simulink model "sistema"  (R2026a)
settings: Solver=ode15s  MaxStep=1E-3
libraries: fl_lib x14, nesl_utility x6, slpidlib x1
settings Model: LastModifiedBy=Mariant Javtech
settings DataIOCC: TimeSaveName=t
settings DebuggingCC: ArtificialAlgebraicLoopMsg=none  MaxConsecutiveZCsMsg=none  OperatingPointInterfaceChecksumMismatchMsg=none
settings SimscapeCC: SimscapeNominalValues="[{\"value\":\"1\",\"unit\":\"A\"},{\"value\":\"1\",\"unit\":\"bar\"},{\"value\":\"1\",\"unit\":\"cm^2\"},{\"value\":\"1\",\"unit\":\"cm^3/s\"},{\"value\":\"1\",\"unit\":\"kJ/kg\"},{\"value\":\"1\",\"unit\":\"kW\"},{\"value\":\"1\",\"unit\":\"l\"},{\"value\":\"1\",\"unit\":\"N\"},{\"value\":\"1\",\"unit\":\"N*m\"},{\"value\":\"1\",\"unit\":\"V\"}]"  SimscapeLogType=none  SimscapeLogDataHistory=5000.0

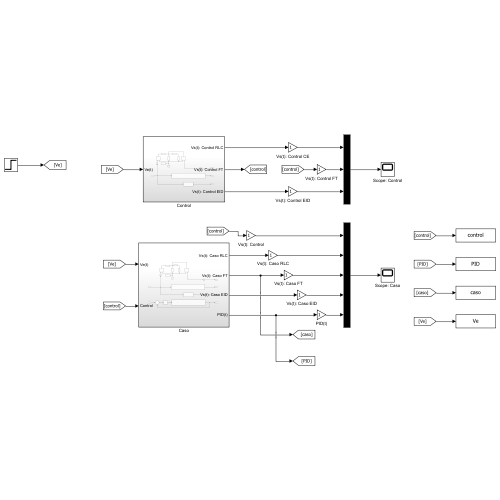
[thumbnail: Simulink's stored preview of the top-level diagram]
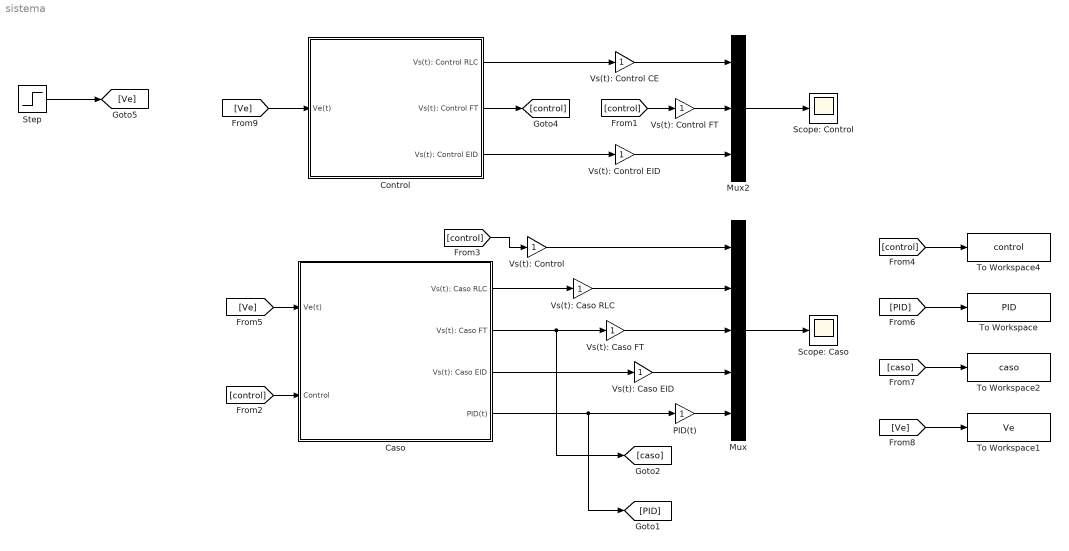
== system sistema ==
  Caso : Subsystem
  Control : Subsystem
  Mux : Mux  Inputs=5
  Mux2 : Mux  Inputs=3
  PID(t) : Gain
  Scope: Caso : Scope
      settings: ActiveDisplayYMinimum=-0.13044665193336266  ActiveDisplayYMaximum=1.1740198674002642
  Scope: Control : Scope
      settings: ActiveDisplayYMinimum=-0.13608  ActiveDisplayYMaximum=1.22472  DataLoggingVariableName=ScopeData2
  Step : Step  Time=0  SampleTime=0
  To Workspace : ToWorkspace  VariableName=PID  SampleTime=-1
  To Workspace1 : ToWorkspace  VariableName=Ve  SampleTime=-1
  To Workspace2 : ToWorkspace  VariableName=caso  SampleTime=-1
  To Workspace4 : ToWorkspace  VariableName=control  SampleTime=-1
  Vs(t): Caso EID : Gain
  Vs(t): Caso FT : Gain
  Vs(t): Caso RLC : Gain
  Vs(t): Control : Gain
  Vs(t): Control CE : Gain
  Vs(t): Control EID : Gain
  Vs(t): Control FT : Gain
  wires:
  Mux/1 -> Scope: Caso/1
  [control] -> Caso/2(Control)
  [control] -> Vs(t): Control/1
  [Ve] -> Caso/1(Ve(t))
  Control/2(Vs(t): Control FT) -> [control]
  Control/1(Vs(t): Control RLC) -> Vs(t): Control CE/1
  Mux2/1 -> Scope: Control/1
  [Ve] -> Control/1(Ve(t))
  Step/1 -> [Ve]
  Vs(t): Control CE/1 -> Mux2/1
  Vs(t): Caso RLC/1 -> Mux/2
  Vs(t): Caso FT/1 -> Mux/3
  [control] -> Vs(t): Control FT/1
  Vs(t): Control FT/1 -> Mux2/2
  Control/3(Vs(t): Control EID) -> Vs(t): Control EID/1
  Vs(t): Control EID/1 -> Mux2/3
  Caso/4(PID(t)) -> [PID], PID(t)/1
  Caso/1(Vs(t): Caso RLC) -> Vs(t): Caso RLC/1
  Caso/2(Vs(t): Caso FT) -> [caso], Vs(t): Caso FT/1
  PID(t)/1 -> Mux/5
  Caso/3(Vs(t): Caso EID) -> Vs(t): Caso EID/1
  Vs(t): Caso EID/1 -> Mux/4
  Vs(t): Control/1 -> Mux/1
  [control] -> To Workspace4/1
  [PID] -> To Workspace/1
  [caso] -> To Workspace2/1
  [Ve] -> To Workspace1/1

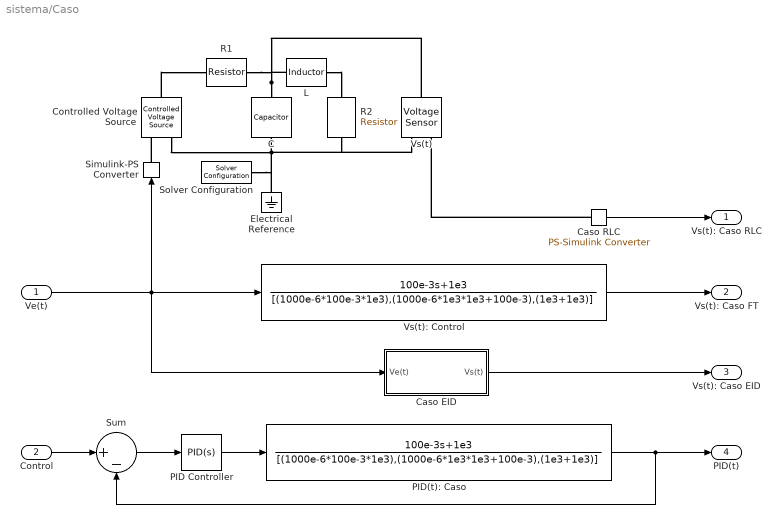
== system sistema/Caso ==
  Ve(t) : Inport
  Control : Inport  Port=2
  C : fl_lib/Electrical/Electrical Elements/Capacitor  c=1000e-6 F  r=1e-6 Ohm  g=0 1/Ohm  i_specify=off  i_priority=None  i=0 A  i_nominal_specify=off  i_nominal_value=1  i_nominal_unit=A  v_specify=off  v_priority=None  v=0 V  v_nominal_specify=off  v_nominal_value=1  v_nominal_unit=V  vc_specify=off  vc_priority=High  vc=0 V  vc_nominal_specify=off  vc_nominal_value=1  vc_nominal_unit=V
  Caso EID : Subsystem
  Caso RLC : nesl_utility/PS-Simulink Converter  PhysicalDomain=network_engine_domain  SubClassName=ps_output  LeftPortType=input  RightPortType=output  PseudoPeriodic=off  Frequencies=[]  VectorFormat=1-D array  Unit=inherit  AffineConversion=off
  Controlled Voltage Source : fl_lib/Electrical/Electrical Sources/Controlled Voltage Source
  Electrical Reference : fl_lib/Electrical/Electrical Elements/Electrical Reference
  L : fl_lib/Electrical/Electrical Elements/Inductor  l=100e-3 H  r=0 Ohm  g=1e-9 1/Ohm  i_specify=off  i_priority=None  i=0 A  i_nominal_specify=off  i_nominal_value=1  i_nominal_unit=A  v_specify=off  v_priority=None  v=0 V  v_nominal_specify=off  v_nominal_value=1  v_nominal_unit=V  i_L_specify=off  i_L_priority=High  i_L=0 A  i_L_nominal_specify=off  i_L_nominal_value=1  i_L_nominal_unit=A
  PID Controller : slpidlib/PID Controller  Controller=PID  Form=Parallel  TimeDomain=Continuous-time  UseExternalTs=off  SampleTime=-1  IntegratorMethod=Forward Euler  FilterMethod=Forward Euler  ControllerParametersSource=internal  P=2048.14768883037  I=776909.685302916  UseKiTs=off  D=0.181141069703887  UseExternalDerivativeSource=off  N=7831.7903058867  UseFilter=on  TunerSelectOption=Transfer Function Based (PID Tuner App)  InitialConditionSource=internal  InitialConditionForIntegrator=0  InitialConditionForFilter=0  DifferentiatorICPrevScaledInput=0  ExternalReset=none  TrackingMode=off  Kt=1  LimitOutput=off  SatLimitsSource=internal  UpperSaturationLimit=inf  LowerSaturationLimit=-inf  LinearizeAsGain=on  AntiWindupMode=none  Kb=1  LimitIntegrator=off  UpperIntegratorSaturationLimit=inf  LowerIntegratorSaturationLimit=-inf  POutMin=[]  POutMax=[]  IOutMin=[]  IOutMax=[]  DOutMin=[]  DOutMax=[]  NOutMin=[]  NOutMax=[]  SumOutMin=[]  SumOutMax=[]  SaturationOutMin=[]  SaturationOutMax=[]  PParamMin=[]  PParamMax=[]  IParamMin=[]  IParamMax=[]  DParamMin=[]  DParamMax=[]  NParamMin=[]  NParamMax=[]  KbParamMin=[]  KbParamMax=[]  KtParamMin=[]  KtParamMax=[]  KbOutMin=[]  KbOutMax=[]  KtOutMin=[]  KtOutMax=[]  IntegratorOutMin=[]  IntegratorOutMax=[]  FilterOutMin=[]  FilterOutMax=[]  SumI1OutMin=[]  SumI1OutMax=[]  SumI2OutMin=[]  SumI2OutMax=[]  SumI3OutMin=[]  SumI3OutMax=[]  SumI4OutMin=[]  SumI4OutMax=[]  SumDOutMin=[]  SumDOutMax=[]  DifferentiatorOutMin=[]  DifferentiatorOutMax=[]  FilterDiffOutCoefMin=[]  FilterDiffOutCoefMax=[]  ReciprocalOutMin=[]  ReciprocalOutMax=[]  SumDenOutMin=[]  SumDenOutMax=[]  SumNumOutMin=[]  SumNumOutMax=[]  DivideOutMin=[]  DivideOutMax=[]  UdiffTsProdOutMin=[]  UdiffTsProdOutMax=[]  NTsProdOutMin=[]  NTsProdOutMax=[]  UintegralTsProdOutMin=[]  UintegralTsProdOutMax=[]  UngainTsProdOutMin=[]  UngainTsProdOutMax=[]  ClampingZeroOutDataTypeStr=Inherit: Inherit via back propagation  ClampingZeroOutMin=[]  ClampingZeroOutMax=[]  FilterDenConstantOutDataTypeStr=Inherit: Inherit via back propagation  FilterDenConstantOutMin=[]  FilterDenConstantOutMax=[]  PCopyOutDataTypeStr=Inherit: Inherit via back propagation  PCopyOutMin=[]  PCopyOutMax=[]  NCopyOutDataTypeStr=Inherit: Inherit via back propagation  NCopyOutMin=[]  NCopyOutMax=[]  IntegratorContinuousStateAttributes=''  IntegratorStateMustResolveToSignalObject=off  IntegratorRTWStateStorageClass=Auto  FilterContinuousStateAttributes=''  FilterStateMustResolveToSignalObject=off  FilterRTWStateStorageClass=Auto  ParallelPVariant=InternalParameters  IdealPVariant=Disabled  IVariant=InternalParameters  DVariant=InternalParameters  IntegratorVariant=Continuous  SatVariant=Disabled  AWVariant=Passthrough  PCopyVariant=Disabled  TRVariant=Disabled  FdbkBlocksVariant=Forward  IdealPFdbkVariant=Disabled  SatFdbkVariant=Disabled  DerivativeFilterVariant=ContFilter  NVariant=InternalParameters  NCopyVariant=Disabled  FilterICVariant=InternalICsFilter  IntegratorICVariant=InternalICs  ExternalResetVariant=Disabled  TRSumVariant=Passthrough  SumFdbkVariant=Disabled  SumVariant=Sum_PID  TsampFilterVariant=InternalTs  TsampNgainVariant=Passthrough  TsampIntegralVariant=Disabled_SignalSpec  ExternalSaturationOutDataTypeStr=Inherit: Same as second input  DerivativeSourceVariant=ErrorSignal  PreIntVariant=InternalPreInt
  PID(t): Caso : TransferFcn  Numerator=[100e-3, 1e3]  Denominator=[(1000e-6*100e-3*1e3),(1000e-6*1e3*1e3+100e-3),(1e3+1e3)]
  R1 : fl_lib/Electrical/Electrical Elements/Resistor  R=1e3 Ohm  i_specify=off  i_priority=None  i=0 A  i_nominal_specify=off  i_nominal_value=1  i_nominal_unit=A  v_specify=off  v_priority=None  v=0 V  v_nominal_specify=off  v_nominal_value=1  v_nominal_unit=V
  R2 : fl_lib/Electrical/Electrical Elements/Resistor  R=1e3 Ohm  i_specify=off  i_priority=None  i=0 A  i_nominal_specify=off  i_nominal_value=1  i_nominal_unit=A  v_specify=off  v_priority=None  v=0 V  v_nominal_specify=off  v_nominal_value=1  v_nominal_unit=V
  Simulink-PS Converter : nesl_utility/Simulink-PS Converter  PhysicalDomain=network_engine_domain  SubClassName=ps_input  LeftPortType=input  RightPortType=output  PseudoPeriodic=off  Frequencies=[]  NoiseDistribution=none  NoiseParameters=[]  Unit=1  AffineConversion=off  FilteringAndDerivatives=provide  SimscapeFilterOrder=1  InputFilterTimeConstant=0.001  UdotUserProvided=0
  Solver Configuration : nesl_utility/Solver Configuration  PhysicalDomain=network_engine_domain  SubClassName=solver  LeftPortType=input  RightPortType=generic  Tones=[]  Harmonics=[]  SimulateNoise=off  Profile=off  UseLocalSampling=off  EnableSwitchedLinearOptims=on  FrequencyDomain=off  UseCCode=off  RelTol=0.001  AbsTol=0.001  MinStep=1e-09  ToWorkspace=off  RevertToSquareIcSolve=off  NumHomotopyIterations=100  PhasorMode=off  PhasorModeNumHarmonics=1  ConsistencySolver=NEWTON_XTOL_AFTER_FTOL  CanonicalOrdering=UNORDERED  OptimizeIntermediates=UNOPTIMIZED  IndexReductionMethod=DerivativeReplacement  DoDC=off  ResidualTolerance=1e-09  ConsistencyTolSource=GLOBAL  ConsistencyAbsTol=0.001  ConsistencyRelTol=0.001  ConsistencyTolFactor=0.001  UseLocalSolver=off  LocalSolverChoice=NE_BACKWARD_EULER_ADVANCER  ResolveIndetEquations=on  FunctionEvalNumThread=1  LocalSolverSampleTime=0.001  DoFixedCost=off  MaxNonlinIter=3  MaxModeIter=2  ComputeImpulses=off  ImpulseIterations=2  LinearAlgebra=auto  LinearAlgebraNumThread=0  EquationFormulation=NE_TIME_EF  DelaysMemoryBudget=1024  AutomaticFiltering=on  FilteringTimeConstant=0.001  PartitionStorageMethod=AS_NEEDED  PartitionMemoryBudget=1024  PartitionMethod=ROBUST  MultibodyUseLocalSolver=off  MultibodyLocalSolverChoice=ODE1  MultibodyLocalSolverSampleTime=0.001
  Sum : Sum  Inputs=|+-
  Vs(t) : fl_lib/Electrical/Electrical Sensors/Voltage Sensor
  Vs(t): Control : TransferFcn  Numerator=[100e-3, 1e3]  Denominator=[(1000e-6*100e-3*1e3),(1000e-6*1e3*1e3+100e-3),(1e3+1e3)]
  Vs(t): Caso RLC : Outport
  Vs(t): Caso FT : Outport  Port=2
  Vs(t): Caso EID : Outport  Port=3
  PID(t) : Outport  Port=4
  wires:
  Sum/1 -> PID Controller/1
  PID(t): Caso/1 -> PID(t)/1, Sum/2
  Control/1 -> Sum/1
  Ve(t)/1 -> Caso EID/1(Ve(t)), Vs(t): Control/1, Simulink-PS Converter/1
  Caso RLC/1 -> Vs(t): Caso RLC/1
  Vs(t): Control/1 -> Vs(t): Caso FT/1
  PID Controller/1 -> PID(t): Caso/1
  Caso EID/1(Vs(t)) -> Vs(t): Caso EID/1
  connections:
  C/LConn1 -- Vs(t)/LConn1 -- R1/LConn1 -- L/LConn1
  C/RConn1 -- Solver Configuration/RConn1 -- Electrical Reference/LConn1 -- Vs(t)/RConn2 -- R2/RConn1 -- Controlled Voltage Source/RConn2
  L/RConn1 -- R2/LConn1
  Controlled Voltage Source/LConn1 -- R1/RConn1
  Simulink-PS Converter/RConn1 -- Controlled Voltage Source/RConn1
  Caso RLC/LConn1 -- Vs(t)/RConn1

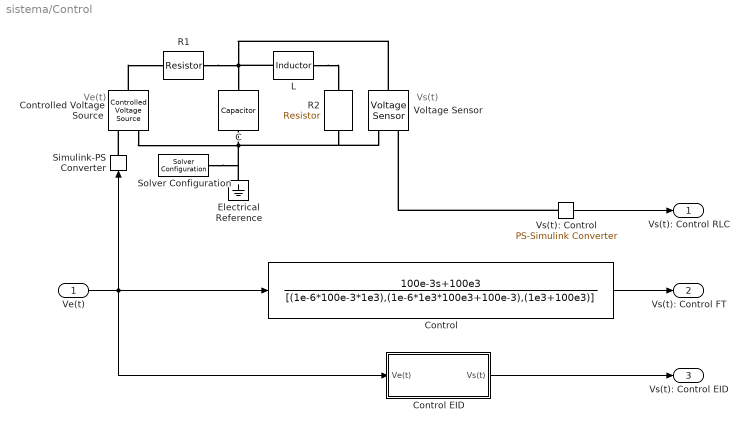
== system sistema/Control ==
  note: Ve(t)
  note: Vs(t)
  Ve(t) : Inport
  C : fl_lib/Electrical/Electrical Elements/Capacitor  c=1e-6 F  r=1e-6 Ohm  g=0 1/Ohm  i_specify=off  i_priority=None  i=0 A  i_nominal_specify=off  i_nominal_value=1  i_nominal_unit=A  v_specify=off  v_priority=None  v=0 V  v_nominal_specify=off  v_nominal_value=1  v_nominal_unit=V  vc_specify=off  vc_priority=High  vc=0 V  vc_nominal_specify=off  vc_nominal_value=1  vc_nominal_unit=V
  Control : TransferFcn  Numerator=[100e-3, 100e3]  Denominator=[(1e-6*100e-3*1e3),(1e-6*1e3*100e3+100e-3),(1e3+100e3)]
  Control EID : Subsystem
  Controlled Voltage Source : fl_lib/Electrical/Electrical Sources/Controlled Voltage Source
  Electrical Reference : fl_lib/Electrical/Electrical Elements/Electrical Reference
  L : fl_lib/Electrical/Electrical Elements/Inductor  l=100e-3 H  r=0 Ohm  g=1e-9 1/Ohm  i_specify=off  i_priority=None  i=0 A  i_nominal_specify=off  i_nominal_value=1  i_nominal_unit=A  v_specify=off  v_priority=None  v=0 V  v_nominal_specify=off  v_nominal_value=1  v_nominal_unit=V  i_L_specify=off  i_L_priority=High  i_L=0 A  i_L_nominal_specify=off  i_L_nominal_value=1  i_L_nominal_unit=A
  R1 : fl_lib/Electrical/Electrical Elements/Resistor  R=1e3 Ohm  i_specify=off  i_priority=None  i=0 A  i_nominal_specify=off  i_nominal_value=1  i_nominal_unit=A  v_specify=off  v_priority=None  v=0 V  v_nominal_specify=off  v_nominal_value=1  v_nominal_unit=V
  R2 : fl_lib/Electrical/Electrical Elements/Resistor  R=100e3 Ohm  i_specify=off  i_priority=None  i=0 A  i_nominal_specify=off  i_nominal_value=1  i_nominal_unit=A  v_specify=off  v_priority=None  v=0 V  v_nominal_specify=off  v_nominal_value=1  v_nominal_unit=V
  Simulink-PS Converter : nesl_utility/Simulink-PS Converter  PhysicalDomain=network_engine_domain  SubClassName=ps_input  LeftPortType=input  RightPortType=output  PseudoPeriodic=off  Frequencies=[]  NoiseDistribution=none  NoiseParameters=[]  Unit=1  AffineConversion=off  FilteringAndDerivatives=provide  SimscapeFilterOrder=1  InputFilterTimeConstant=0.001  UdotUserProvided=0
  Solver Configuration : nesl_utility/Solver Configuration  PhysicalDomain=network_engine_domain  SubClassName=solver  LeftPortType=input  RightPortType=generic  Tones=[]  Harmonics=[]  SimulateNoise=off  Profile=off  UseLocalSampling=off  EnableSwitchedLinearOptims=on  FrequencyDomain=off  UseCCode=off  RelTol=0.001  AbsTol=0.001  MinStep=1e-09  ToWorkspace=off  RevertToSquareIcSolve=off  NumHomotopyIterations=100  PhasorMode=off  PhasorModeNumHarmonics=1  ConsistencySolver=NEWTON_XTOL_AFTER_FTOL  CanonicalOrdering=UNORDERED  OptimizeIntermediates=UNOPTIMIZED  IndexReductionMethod=DerivativeReplacement  DoDC=off  ResidualTolerance=1e-09  ConsistencyTolSource=GLOBAL  ConsistencyAbsTol=0.001  ConsistencyRelTol=0.001  ConsistencyTolFactor=0.001  UseLocalSolver=off  LocalSolverChoice=NE_BACKWARD_EULER_ADVANCER  ResolveIndetEquations=on  FunctionEvalNumThread=1  LocalSolverSampleTime=0.001  DoFixedCost=off  MaxNonlinIter=3  MaxModeIter=2  ComputeImpulses=off  ImpulseIterations=2  LinearAlgebra=auto  LinearAlgebraNumThread=0  EquationFormulation=NE_TIME_EF  DelaysMemoryBudget=1024  AutomaticFiltering=on  FilteringTimeConstant=0.001  PartitionStorageMethod=AS_NEEDED  PartitionMemoryBudget=1024  PartitionMethod=ROBUST  MultibodyUseLocalSolver=off  MultibodyLocalSolverChoice=ODE1  MultibodyLocalSolverSampleTime=0.001
  Voltage Sensor : fl_lib/Electrical/Electrical Sensors/Voltage Sensor
  Vs(t): Control : nesl_utility/PS-Simulink Converter  PhysicalDomain=network_engine_domain  SubClassName=ps_output  LeftPortType=input  RightPortType=output  PseudoPeriodic=off  Frequencies=[]  VectorFormat=1-D array  Unit=inherit  AffineConversion=off
  Vs(t): Control RLC : Outport
  Vs(t): Control FT : Outport  Port=2
  Vs(t): Control EID : Outport  Port=3
  wires:
  Control/1 -> Vs(t): Control FT/1
  Vs(t): Control/1 -> Vs(t): Control RLC/1
  Ve(t)/1 -> Control EID/1(Ve(t)), Control/1, Simulink-PS Converter/1
  Control EID/1(Vs(t)) -> Vs(t): Control EID/1
  connections:
  Simulink-PS Converter/RConn1 -- Controlled Voltage Source/RConn1
  Vs(t): Control/LConn1 -- Voltage Sensor/RConn1
  Controlled Voltage Source/LConn1 -- R1/RConn1
  R1/LConn1 -- Voltage Sensor/LConn1 -- L/LConn1 -- C/LConn1
  Controlled Voltage Source/RConn2 -- Solver Configuration/RConn1 -- Electrical Reference/LConn1 -- Voltage Sensor/RConn2 -- R2/RConn1 -- C/RConn1
  L/RConn1 -- R2/LConn1

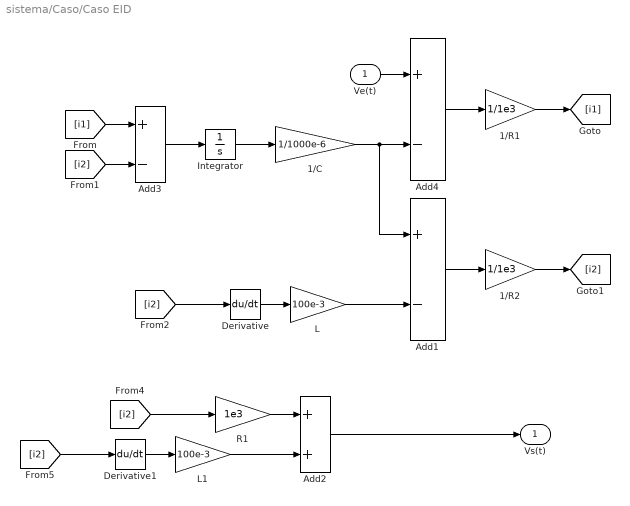
== system sistema/Caso/Caso EID ==
  Ve(t) : Inport
  1/C : Gain  Gain=1/1000e-6
  1/R1 : Gain  Gain=1/1e3
  1/R2 : Gain  Gain=1/1e3
  Add1 : Sum  Inputs=+-
  Add2 : Sum
  Add3 : Sum  Inputs=+-
  Add4 : Sum  Inputs=+-
  Derivative : Derivative
  Derivative1 : Derivative
  Integrator : Integrator
  L : Gain  Gain=100e-3
  L1 : Gain  Gain=100e-3
  R1 : Gain  Gain=1e3
  Vs(t) : Outport
  wires:
  [i1] -> Add3/1
  [i2] -> Add3/2
  Add3/1 -> Integrator/1
  Integrator/1 -> 1/C/1
  1/C/1 -> Add1/1, Add4/2
  Ve(t)/1 -> Add4/1
  Add4/1 -> 1/R1/1
  1/R1/1 -> [i1]
  Add1/1 -> 1/R2/1
  1/R2/1 -> [i2]
  L/1 -> Add1/2
  Derivative/1 -> L/1
  [i2] -> Derivative/1
  [i2] -> Derivative1/1
  L1/1 -> Add2/2
  R1/1 -> Add2/1
  Derivative1/1 -> L1/1
  [i2] -> R1/1
  Add2/1 -> Vs(t)/1

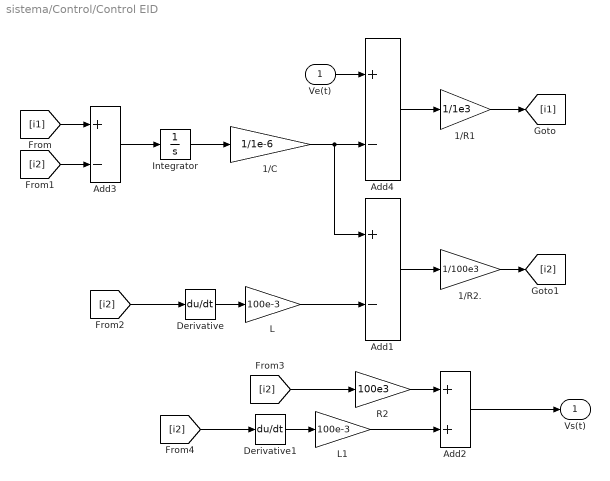
== system sistema/Control/Control EID ==
  Ve(t) : Inport
  1/C : Gain  Gain=1/1e-6
  1/R1 : Gain  Gain=1/1e3
  1/R2. : Gain  Gain=1/100e3
  Add1 : Sum  Inputs=+-
  Add2 : Sum
  Add3 : Sum  Inputs=+-
  Add4 : Sum  Inputs=+-
  Derivative : Derivative
  Derivative1 : Derivative
  Integrator : Integrator
  L : Gain  Gain=100e-3
  L1 : Gain  Gain=100e-3
  R2 : Gain  Gain=100e3
  Vs(t) : Outport
  wires:
  [i2] -> Derivative/1
  1/R2./1 -> [i2]
  [i2] -> R2/1
  1/R1/1 -> [i1]
  L/1 -> Add1/2
  Add1/1 -> 1/R2./1
  1/C/1 -> Add1/1, Add4/2
  Add3/1 -> Integrator/1
  [i2] -> Add3/2
  [i1] -> Add3/1
  Integrator/1 -> 1/C/1
  Derivative/1 -> L/1
  Add4/1 -> 1/R1/1
  Ve(t)/1 -> Add4/1
  R2/1 -> Add2/1
  Add2/1 -> Vs(t)/1
  L1/1 -> Add2/2
  Derivative1/1 -> L1/1
  [i2] -> Derivative1/1
